simulink model "elec_mech"  (R2023a)
settings: Solver=VariableStepAuto  StartTime=0.0  StopTime=10.0  RelTol=1e-3
libraries: fl_lib x27, nesl_utility x11
settings Model: Creator=ahmad  LastModifiedBy=ahmad

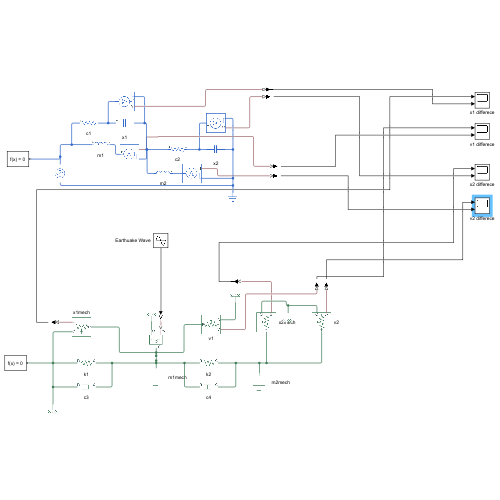
[thumbnail: Simulink's stored preview of the top-level diagram]
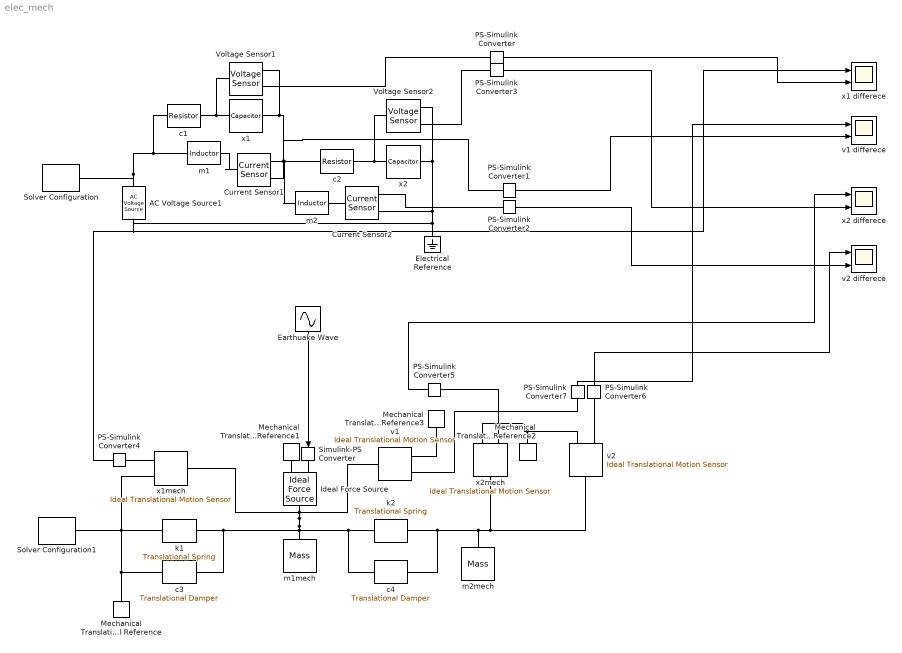
== system elec_mech ==
  AC Voltage Source1 : fl_lib/Electrical/Electrical Sources/AC Voltage Source  amp=5000 V  shift=0 deg  frequency=4 Hz  omega=0 rad/s
  Current Sensor1 : fl_lib/Electrical/Electrical Sensors/Current Sensor
  Current Sensor2 : fl_lib/Electrical/Electrical Sensors/Current Sensor
  Earthuake Wave : Sin  Amplitude=5000  Frequency=8*pi  SampleTime=0
  Electrical Reference : fl_lib/Electrical/Electrical Elements/Electrical Reference
  Ideal Force Source : fl_lib/Mechanical/Mechanical Sources/Ideal Force Source
  Mechanical Translational Reference{,1..3} (4 alike) : fl_lib/Mechanical/Translational Elements/Mechanical Translational Reference
  PS-Simulink Converter{,1..7} (8 alike) : nesl_utility/PS-Simulink Converter  PhysicalDomain=network_engine_domain  SubClassName=ps_output  LeftPortType=input  RightPortType=output  PseudoPeriodic=off  Frequencies=[]  VectorFormat=inherit  Unit=inherit  AffineConversion=off
  Simulink-PS Converter : nesl_utility/Simulink-PS Converter  PhysicalDomain=network_engine_domain  SubClassName=ps_input  LeftPortType=input  RightPortType=output  PseudoPeriodic=off  Frequencies=[]  NoiseDistribution=none  NoiseParameters=[]  Unit=1  AffineConversion=off  FilteringAndDerivatives=provide  SimscapeFilterOrder=1  InputFilterTimeConstant=0.001  UdotUserProvided=0
  Solver Configuration : nesl_utility/Solver Configuration  PhysicalDomain=network_engine_domain  SubClassName=solver  LeftPortType=input  RightPortType=generic  Tones=[]  Harmonics=[]  SimulateNoise=off  Profile=off  UseLocalSampling=off  EnableSwitchedLinearOptims=on  FrequencyDomain=off  UseCCode=off  RelTol=0.001  AbsTol=0.001  MinStep=1e-09  ToWorkspace=off  RevertToSquareIcSolve=off  NumHomotopyIterations=100  PhasorMode=off  PhasorModeNumHarmonics=1  ConsistencySolver=NEWTON_XTOL_AFTER_FTOL  IndexReductionMethod=DerivativeReplacement  DoDC=off  ResidualTolerance=1e-09  ConsistencyTolSource=GLOBAL  ConsistencyAbsTol=0.001  ConsistencyRelTol=0.001  ConsistencyTolFactor=0.001  UseLocalSolver=off  LocalSolverChoice=NE_BACKWARD_EULER_ADVANCER  ResolveIndetEquations=on  FunctionEvalNumThread=1  LocalSolverSampleTime=0.001  DoFixedCost=off  MaxNonlinIter=3  MaxModeIter=2  ComputeImpulses=off  ImpulseIterations=2  LinearAlgebra=auto  LinearAlgebraNumThread=0  EquationFormulation=NE_TIME_EF  DelaysMemoryBudget=1024  AutomaticFiltering=on  FilteringTimeConstant=0.001  PartitionStorageMethod=AS_NEEDED  PartitionMemoryBudget=1024  PartitionMethod=ROBUST
  Solver Configuration1 : nesl_utility/Solver Configuration  PhysicalDomain=network_engine_domain  SubClassName=solver  LeftPortType=input  RightPortType=generic  Tones=[]  Harmonics=[]  SimulateNoise=off  Profile=off  UseLocalSampling=off  EnableSwitchedLinearOptims=on  FrequencyDomain=off  UseCCode=off  RelTol=0.001  AbsTol=0.001  MinStep=1e-09  ToWorkspace=off  RevertToSquareIcSolve=off  NumHomotopyIterations=100  PhasorMode=off  PhasorModeNumHarmonics=1  ConsistencySolver=NEWTON_XTOL_AFTER_FTOL  IndexReductionMethod=DerivativeReplacement  DoDC=off  ResidualTolerance=1e-09  ConsistencyTolSource=GLOBAL  ConsistencyAbsTol=0.001  ConsistencyRelTol=0.001  ConsistencyTolFactor=0.001  UseLocalSolver=off  LocalSolverChoice=NE_BACKWARD_EULER_ADVANCER  ResolveIndetEquations=on  FunctionEvalNumThread=1  LocalSolverSampleTime=0.001  DoFixedCost=off  MaxNonlinIter=3  MaxModeIter=2  ComputeImpulses=off  ImpulseIterations=2  LinearAlgebra=auto  LinearAlgebraNumThread=0  EquationFormulation=NE_TIME_EF  DelaysMemoryBudget=1024  AutomaticFiltering=on  FilteringTimeConstant=0.001  PartitionStorageMethod=AS_NEEDED  PartitionMemoryBudget=1024  PartitionMethod=ROBUST
  Voltage Sensor1 : fl_lib/Electrical/Electrical Sensors/Voltage Sensor
  Voltage Sensor2 : fl_lib/Electrical/Electrical Sensors/Voltage Sensor
  c1 : fl_lib/Electrical/Electrical Elements/Resistor  R=4 MOhm  i_specify=off  i_priority=None  i=0 A  i_nominal_specify=off  i_nominal_unit=A  i_nominal_value=1  v_specify=off  v_priority=None  v=0 V  v_nominal_specify=off  v_nominal_unit=V  v_nominal_value=1
  c2 : fl_lib/Electrical/Electrical Elements/Resistor  R=2 MOhm  i_specify=off  i_priority=None  i=0 A  i_nominal_specify=off  i_nominal_unit=A  i_nominal_value=1  v_specify=off  v_priority=None  v=0 V  v_nominal_specify=off  v_nominal_unit=V  v_nominal_value=1
  c3 : fl_lib/Mechanical/Translational Elements/Translational Damper  D=4e6 N*s/m  v_specify=on  v_priority=None  v=0 m/s  v_nominal_specify=off  v_nominal_unit=m/s  v_nominal_value=1  f_specify=off  f_priority=None  f=0 N  f_nominal_specify=off  f_nominal_unit=N  f_nominal_value=1
  c4 : fl_lib/Mechanical/Translational Elements/Translational Damper  D=2e6 N*s/m  v_specify=on  v_priority=None  v=0 m/s  v_nominal_specify=off  v_nominal_unit=m/s  v_nominal_value=1  f_specify=off  f_priority=None  f=0 N  f_nominal_specify=off  f_nominal_unit=N  f_nominal_value=1
  k1 : fl_lib/Mechanical/Translational Elements/Translational Spring  spr_rate=4e6 N/m  v_specify=off  v_priority=None  v=0 m/s  v_nominal_specify=off  v_nominal_unit=m/s  v_nominal_value=1  f_specify=off  f_priority=None  f=0 N  f_nominal_specify=off  f_nominal_unit=N  f_nominal_value=1  x_specify=on  x_priority=High  x=0 m  x_nominal_specify=off  x_nominal_unit=m  x_nominal_value=1
  k2 : fl_lib/Mechanical/Translational Elements/Translational Spring  spr_rate=2e5 N/m  v_specify=off  v_priority=None  v=0 m/s  v_nominal_specify=off  v_nominal_unit=m/s  v_nominal_value=1  f_specify=off  f_priority=None  f=0 N  f_nominal_specify=off  f_nominal_unit=N  f_nominal_value=1  x_specify=on  x_priority=High  x=0 m  x_nominal_specify=off  x_nominal_unit=m  x_nominal_value=1
  m1 : fl_lib/Electrical/Electrical Elements/Inductor  l=4000 H  r=0 Ohm  g=0 1/Ohm  i_specify=on  i_priority=None  i=0 A  i_nominal_specify=off  i_nominal_unit=A  i_nominal_value=1  v_specify=off  v_priority=None  v=0 V  v_nominal_specify=off  v_nominal_unit=V  v_nominal_value=1  i_L_specify=off  i_L_priority=High  i_L=0 A  i_L_nominal_specify=off  i_L_nominal_unit=A  i_L_nominal_value=1
  m1mech : fl_lib/Mechanical/Translational Elements/Mass  mass=4000 kg  num_ports=foundation.enum.numPorts2.one  v_specify=off  v_priority=High  v=0 m/s  v_nominal_specify=off  v_nominal_unit=m/s  v_nominal_value=1  f_specify=off  f_priority=None  f=0 N  f_nominal_specify=off  f_nominal_unit=N  f_nominal_value=1
  m2 : fl_lib/Electrical/Electrical Elements/Inductor  l=200 H  r=0 Ohm  g=0 1/Ohm  i_specify=on  i_priority=None  i=0 A  i_nominal_specify=off  i_nominal_unit=A  i_nominal_value=1  v_specify=off  v_priority=None  v=0 V  v_nominal_specify=off  v_nominal_unit=V  v_nominal_value=1  i_L_specify=off  i_L_priority=High  i_L=0 A  i_L_nominal_specify=off  i_L_nominal_unit=A  i_L_nominal_value=1
  m2mech : fl_lib/Mechanical/Translational Elements/Mass  mass=200 kg  num_ports=foundation.enum.numPorts2.one  v_specify=off  v_priority=High  v=0 m/s  v_nominal_specify=off  v_nominal_unit=m/s  v_nominal_value=1  f_specify=off  f_priority=None  f=0 N  f_nominal_specify=off  f_nominal_unit=N  f_nominal_value=1
  v1 : fl_lib/Mechanical/Mechanical Sensors/Ideal Translational Motion Sensor  reference=foundation.enum.MeasurementReference.difference  acceleration_port=false  velocity_port=true  position_port=false  offset=0 m
      settings: InternalSimscapePortConfiguration="{\"Bottom\":[],\"Left\":[{\"id\":\"R\",\"label\":\"R\",\"type\":\"foundation.mechanical.translational.translational\"}],\"Right\":[{\"id\":\"C\",\"label\":\"C\",\"type\":\"foundation.mechanical.translational.translational\"},{\"id\":\"V\",\"label\":\"V\",\"type\":\"output\"}],\"Top\":[]}"
  v1 differece : Scope  NumInputPorts=2
  v2 : fl_lib/Mechanical/Mechanical Sensors/Ideal Translational Motion Sensor  reference=foundation.enum.MeasurementReference.difference  acceleration_port=false  velocity_port=true  position_port=false  offset=0 m
      settings: InternalSimscapePortConfiguration="{\"Bottom\":[],\"Left\":[{\"id\":\"R\",\"label\":\"R\",\"type\":\"foundation.mechanical.translational.translational\"}],\"Right\":[{\"id\":\"C\",\"label\":\"C\",\"type\":\"foundation.mechanical.translational.translational\"},{\"id\":\"V\",\"label\":\"V\",\"type\":\"output\"}],\"Top\":[]}"
  v2 differece : Scope  NumInputPorts=2
  x1 : fl_lib/Electrical/Electrical Elements/Capacitor  c=0.25 uF  r=0 Ohm  g=0 1/Ohm  i_specify=off  i_priority=None  i=0 A  i_nominal_specify=off  i_nominal_unit=A  i_nominal_value=1  v_specify=on  v_priority=None  v=0 V  v_nominal_specify=off  v_nominal_unit=V  v_nominal_value=1  vc_specify=off  vc_priority=High  vc=0 V  vc_nominal_specify=off  vc_nominal_unit=V  vc_nominal_value=1
  x1 differece : Scope  NumInputPorts=2
  x1mech : fl_lib/Mechanical/Mechanical Sensors/Ideal Translational Motion Sensor  reference=foundation.enum.MeasurementReference.difference  acceleration_port=false  velocity_port=false  position_port=true  offset=0 m
      settings: InternalSimscapePortConfiguration="{\"Bottom\":[],\"Left\":[{\"id\":\"R\",\"label\":\"R\",\"type\":\"foundation.mechanical.translational.translational\"}],\"Right\":[{\"id\":\"C\",\"label\":\"C\",\"type\":\"foundation.mechanical.translational.translational\"},{\"id\":\"P\",\"label\":\"P\",\"type\":\"output\"}],\"Top\":[]}"
  x2 : fl_lib/Electrical/Electrical Elements/Capacitor  c=5 uF  r=0 Ohm  g=0 1/Ohm  i_specify=off  i_priority=None  i=0 A  i_nominal_specify=off  i_nominal_unit=A  i_nominal_value=1  v_specify=on  v_priority=None  v=0 V  v_nominal_specify=off  v_nominal_unit=V  v_nominal_value=1  vc_specify=off  vc_priority=High  vc=0 V  vc_nominal_specify=off  vc_nominal_unit=V  vc_nominal_value=1
  x2 differece : Scope  NumInputPorts=2
  x2mech : fl_lib/Mechanical/Mechanical Sensors/Ideal Translational Motion Sensor  reference=foundation.enum.MeasurementReference.difference  acceleration_port=false  velocity_port=false  position_port=true  offset=0 m
      settings: InternalSimscapePortConfiguration="{\"Bottom\":[],\"Left\":[{\"id\":\"R\",\"label\":\"R\",\"type\":\"foundation.mechanical.translational.translational\"}],\"Right\":[{\"id\":\"C\",\"label\":\"C\",\"type\":\"foundation.mechanical.translational.translational\"},{\"id\":\"P\",\"label\":\"P\",\"type\":\"output\"}],\"Top\":[]}"
  wires:
  PS-Simulink Converter2/1 -> v2 differece/2
  PS-Simulink Converter/1 -> x1 differece/2
  PS-Simulink Converter1/1 -> v1 differece/2
  PS-Simulink Converter3/1 -> x2 differece/2
  PS-Simulink Converter4/1 -> x1 differece/1
  PS-Simulink Converter7/1 -> v1 differece/1
  Earthuake Wave/1 -> Simulink-PS Converter/1
  PS-Simulink Converter5/1 -> x2 differece/1
  PS-Simulink Converter6/1 -> v2 differece/1
  connections:
  x2/LConn1 -- c2/RConn1 -- Voltage Sensor2/LConn1
  c1/RConn1 -- x1/LConn1 -- Voltage Sensor1/LConn1
  Current Sensor1/RConn2 -- x1/RConn1 -- Voltage Sensor1/RConn2 -- m2/LConn1 -- c2/LConn1
  x2/RConn1 -- Current Sensor2/RConn2 -- AC Voltage Source1/RConn1 -- Electrical Reference/LConn1 -- Voltage Sensor2/RConn2
  m1/LConn1 -- c1/LConn1 -- Solver Configuration/RConn1 -- AC Voltage Source1/LConn1
  Current Sensor2/RConn1 -- PS-Simulink Converter2/LConn1
  Voltage Sensor2/RConn1 -- PS-Simulink Converter3/LConn1
  Current Sensor2/LConn1 -- m2/RConn1
  Current Sensor1/RConn1 -- PS-Simulink Converter1/LConn1
  Current Sensor1/LConn1 -- m1/RConn1
  Voltage Sensor1/RConn1 -- PS-Simulink Converter/LConn1
  x2mech/LConn1 -- k2/RConn1 -- c4/RConn1 -- m2mech/LConn1 -- v2/LConn1
  Mechanical Translational Reference2/LConn1 -- x2mech/RConn1 -- v2/RConn1
  k2/LConn1 -- c4/LConn1 -- v1/LConn1 -- x1mech/LConn1 -- Ideal Force Source/LConn1 -- m1mech/LConn1 -- k1/RConn1 -- c3/RConn1
  k1/LConn1 -- Mechanical Translational Reference/LConn1 -- c3/LConn1 -- Solver Configuration1/RConn1 -- x1mech/RConn1
  Simulink-PS Converter/RConn1 -- Ideal Force Source/RConn1
  v2/RConn2 -- PS-Simulink Converter6/LConn1
  v1/RConn2 -- PS-Simulink Converter7/LConn1
  PS-Simulink Converter4/LConn1 -- x1mech/RConn2
  v1/RConn1 -- Mechanical Translational Reference3/LConn1
  x2mech/RConn2 -- PS-Simulink Converter5/LConn1
  Mechanical Translational Reference1/LConn1 -- Ideal Force Source/RConn2
